simulink model "CLLCTestHarnessPlant"  (R2026a)
settings: Solver=ode23t  StopTime=5e-3  FixedStep=1e-4  MaxStep=1e-6  AbsTol=1e-3
PreLoadFcn:
  | CLLCConverterDefaultInputParameters;
undefined symbols (not defined in the file or in its folder): CLLCCompensator, CLLCController, CLLCDesign, DiscIntNeverNeededParam
libraries: fl_lib x46, nesl_utility x45, ee_lib x35
(part 1 of 4)
Description:
  | Design of LLC Resonant Converter
settings Model: ExtModeTrigDuration=100  Creator=The MathWorks, Inc.  LastModifiedBy=vsolaise
settings SolverCC: MaxConsecutiveMinStep=10
settings DataIOCC: StateSaveName=tmp_raccel_xout  SignalLoggingName=logsoutCLLCConverter  OutputTimes=[0:1.1*3*Voc/(1*2000):1.1*3*Voc/1]
settings OptimizationCC: EfficientMapNaN2IntZero=off
settings HardwareCC: ProdHWDeviceType=Intel->x86-32 (Windows32)  TargetBitPerPointer=64.0  TargetBitPerSizeT=64.0  TargetBitPerPtrDiffT=64.0  TargetLongLongMode=on  TargetIntDivRoundTo=Zero  TargetEndianess=LittleEndian  TargetWordSize=64.0  TargetHWDeviceType=MATLAB Host  ProdEqTarget=off
settings RTWCC: SystemTargetFile=raccel.tlc  TemplateMakefile=raccel_default_tmf  RTWVerbose=off  RTWUseSimCustomCode=on
settings CodeAppCC: GenerateComments=off  MaxIdLength=128.0  SimulinkBlockComments=off
settings RaccelTargetCC: ExtModeTransport=0.0  ExtModeStaticAllocSize=1000000.0  ENABLE_SLEXEC_SSBRIDGE=1.0  RTWCAPIParams=on  RTWCAPIRootIO=on  MultiwordLength=2048.0
settings SimscapeCC: SimscapeNominalValues="[{\"value\":\"1\",\"unit\":\"A\"},{\"value\":\"1\",\"unit\":\"bar\"},{\"value\":\"1\",\"unit\":\"cm^2\"},{\"value\":\"1\",\"unit\":\"cm^3/s\"},{\"value\":\"1\",\"unit\":\"kJ/kg\"},{\"value\":\"1\",\"unit\":\"kW\"},{\"value\":\"1\",\"unit\":\"l\"},{\"value\":\"1\",\"unit\":\"N\"},{\"value\":\"1\",\"unit\":\"N*m\"},{\"value\":\"1\",\"unit\":\"V\"}]"  SimscapeLogName=SimlogCLLCConverter  SimscapeLogLimitData=off  SimscapeLogDataHistory=5000.0

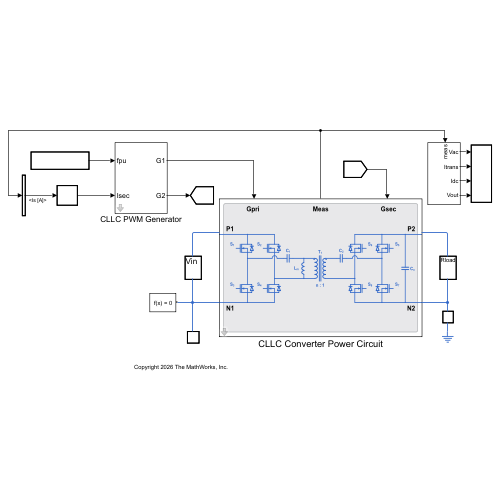
[thumbnail: Simulink's stored preview of the top-level diagram]
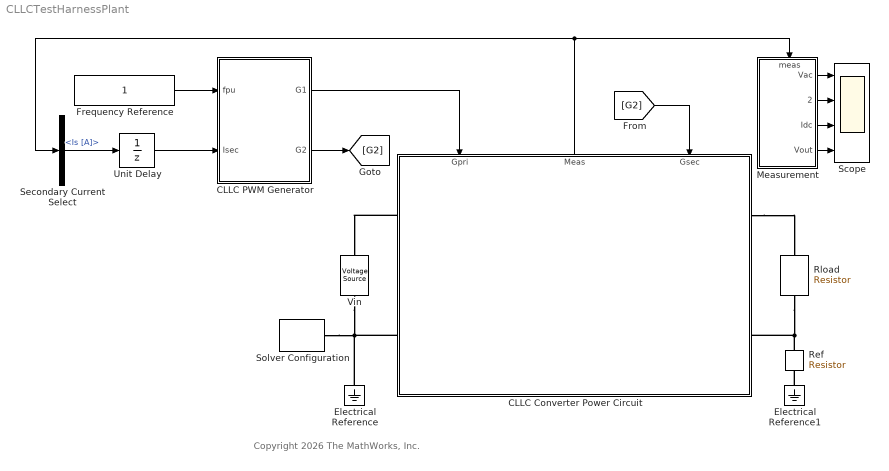
== system CLLCTestHarnessPlant ==
  note: Copyright 2026 The MathWorks, Inc.
  CLLC Converter Power Circuit : Subsystem  mask(CLLC Converter Plant){modelOption=Detailed, C1=6.9269e-7, C1_unit=F, Rcr1=0.001, Rcr1_unit=Ohm, C2=7.487e-7, C2_unit=F, Rcr2=0.001, Rcr2_unit=Ohm, Llk1=3.6568e-6, Llk1_unit=H, R1=0.01, R1_unit=Ohm, Llk2=3.3829e-6, Llk2_unit=H, R2=0.01, R2_unit=Ohm, Lm=5.4852e-5, Lm_unit=H, N1=30, N2=29, Co=1.0667e-3, Co_unit=F, Rco=0.02, Rco_unit=Ohm, Vco=350, Vco_unit=V, PrimaryDeviceOption=Ideal Switch, PrimaryRon=0.0001, PrimaryRon_unit=Ohm, PrimaryGoff=1e-5, PrimaryGoff_unit=1/Ohm, PrimaryVth=2.5, PrimaryVth_unit=V, PrimaryVbodydiodeOn=0.6, PrimaryVbodydiodeOn_unit=V, PrimaryRbodydiodeOn=0.0001, PrimaryRbodydiodeOn_unit=Ohm, PrimaryGbodydiodeOff=1e-5, PrimaryGbodydiodeOff_unit=1/Ohm, PrimaryCparasitic=2e-10, PrimaryCparasitic_unit=F, SecondaryDeviceOption=Ideal Switch, SecondaryRon=0.0001, SecondaryRon_unit=Ohm, SecondaryGoff=1e-5, SecondaryGoff_unit=1/Ohm, SecondaryVth=2.5, SecondaryVth_unit=V, SecondaryVbodydiodeOn=0.6, SecondaryVbodydiodeOn_unit=V, SecondaryRbodydiodeOn=0.0001, SecondaryRbodydiodeOn_unit=Ohm, SecondaryGbodydiodeOff=1e-5, SecondaryGbodydiodeOff_unit=1/Ohm, SecondaryCparasitic=2e-10, SecondaryCparasitic_unit=F, PrimarySimTemp=25, PrimarySimTemp_unit=degC, SecondarySimTemp=25, SecondarySimTemp_unit=degC}
      mask prompts: modelOption "Model option"; C1 "Primary resonant capacitance (C1)"; Rcr1 "Primary resonant capacitor ESR (Rcr1)"; C2 "Secondary resonant capacitance (C2)"; Rcr2 "Secondary resonant capacitor ESR (Rcr2)"; Llk1 "Primary leakage inductance (Llk1)"; R1 "Primary resistance (R1)"; Llk2 "Secondary leakage inductance (Llk2)"; R2 "Secondary resistance (R2)"; Lm "Magnetizing inductance (Lm)"; N1 "Transformer primary number of turns (N1)"; N2 "Transformer secondary number of turns (N2)"; Co "Secondary output capacitance (Co)"; Rco "Secondary output capacitance ESR (Rco)"; Vco "Initial output capacitor voltage"; PrimaryDeviceOption "Select the primary switching device"; PrimaryRon "On-state resistance"; PrimaryGoff "Off-state conductance"; PrimaryVth "Threshold voltage"; PrimaryVbodydiodeOn "Body diode forward voltage"; PrimaryRbodydiodeOn "Body diode on-resistance"; PrimaryGbodydiodeOff "Body diode off-conductance"; PrimaryCparasitic "MOSFET parasitic capacitance"; SecondaryDeviceOption "Select the secondary switching device"; SecondaryRon "On-state resistance"; SecondaryGoff "Off-state conductance"; SecondaryVth "Threshold voltage"; SecondaryVbodydiodeOn "Body diode forward voltage"; SecondaryRbodydiodeOn "Body diode on-resistance"; SecondaryGbodydiodeOff "Body diode off-conductance"; SecondaryCparasitic "MOSFET parasitic capacitance"; PrimarySimTemp "Simulation temperature"; SecondarySimTemp "Simulation temperature"
      mask help: This block models the power circuit of the CLLC resonant converter. You can choose between different semicondcutor switch model for primary and secondaryconverter. You can choose between ideal semiconductor switch, MOSFET without thermal port and tabulated MOSFET with thermal port.
      mask init:
      | %% Unit conversion: convert displayed values to base SI units
      | convMap = containers.Map( ...
      |     {'W','kW','MW','V','kV','mV','F','mF','uF','nF','pF', ...
      |      'H','mH','uH','nH','Ohm','kOhm','mOhm','S','mS','1/Ohm'}, ...
      |     {1, 1e3, 1e6, 1, 1e3, 1e-3, 1, 1e-3, 1e-6, 1e-9, 1e-12, ...
      |      1, 1e-3, 1e-6, 1e-9, 1, 1e3, 1e-3, 1, 1e-3, 1});
      | C1 = C1 * convMap(C1_unit);
      | Rcr1 = Rcr1 * convMap(Rcr1_unit);
      | C2 = C2 * convMap(C2_unit);
      | Rcr2 = Rcr2 * convMap(Rcr2_unit);
      | Llk1 = Llk1 * convMap(Llk1_unit);
      | R1 = R1 * convMap(R1_unit);
      | Llk2 = Llk2 * convMap(Llk2_unit);
      | R2 = R2 * convMap(R2_unit);
      | Lm = Lm * convMap(Lm_unit);
      | Co = Co * convMap(Co_unit);
      | Rco = Rco * convMap(Rco_unit);
      | Vco = Vco * convMap(Vco_unit);
      | PrimaryRon = PrimaryRon * convMap(PrimaryRon_unit);
      | PrimaryGoff = PrimaryGoff * convMap(PrimaryGoff_unit);
      | PrimaryVth = PrimaryVth * convMap(PrimaryVth_unit);
      | PrimaryVbodydiodeOn = PrimaryVbodydiodeOn * convMap(PrimaryVbodydiodeOn_unit);
      | PrimaryRbodydiodeOn = PrimaryRbodydiodeOn * convMap(PrimaryRbodydiodeOn_unit);
      | PrimaryGbodydiodeOff = PrimaryGbodydiodeOff * convMap(PrimaryGbodydiodeOff_unit);
      | PrimaryCparasitic = PrimaryCparasitic * convMap(PrimaryCparasitic_unit);
      | SecondaryRon = SecondaryRon * convMap(SecondaryRon_unit);
      | SecondaryGoff = SecondaryGoff * convMap(SecondaryGoff_unit);
      | SecondaryVth = SecondaryVth * convMap(SecondaryVth_unit);
      | SecondaryVbodydiodeOn = SecondaryVbodydiodeOn * convMap(SecondaryVbodydiodeOn_unit);
      | SecondaryRbodydiodeOn = SecondaryRbodydiodeOn * convMap(SecondaryRbodydiodeOn_unit);
      | SecondaryGbodydiodeOff = SecondaryGbodydiodeOff * convMap(SecondaryGbodydiodeOff_unit);
      | SecondaryCparasitic = SecondaryCparasitic * convMap(SecondaryCparasitic_unit);
      | % Simulation temperature (primary bridge, thermal MOSFETs)
      | % Temperature is an OFFSET unit (K = degC + 273.15), so it cannot use the
      | % multiplicative convMap above; convert it explicitly. PrimarySimTemp_K is read directly
      | % by each primary thermal MOSFET junction-temperature initial target and by every
      | % Temperature Source in the primary bridge.
      | if strcmp(PrimarySimTemp_unit, 'degC')
      |     PrimarySimTemp_K = PrimarySimTemp + 273.15;
      | elseif strcmp(PrimarySimTemp_unit, 'K')
      |     PrimarySimTemp_K = PrimarySimTemp;
      | else
      |     error('CLLC Converter Power Circuit: unrecognized simulation-temperature unit "%s" (expected degC or K).', PrimarySimTemp_unit);
      | end
      | % Simulation temperature (secondary bridge, thermal MOSFETs)
      | % Temperature is an OFFSET unit (K = degC + 273.15), so it cannot use the
      | % multiplicative convMap above; convert it explicitly. SecondarySimTemp_K is read directly
      | % by each secondary thermal MOSFET junction-temperature initial target and by every
      | % Temperature Source in the secondary bridge.
      | if strcmp(SecondarySimTemp_unit, 'degC')
      |     SecondarySimTemp_K = SecondarySimTemp + 273.15;
      | elseif strcmp(SecondarySimTemp_unit, 'K')
      |     SecondarySimTemp_K = SecondarySimTemp;
      | else
      |     error('CLLC Converter Power Circuit: unrecognized simulation-temperature unit "%s" (expected degC or K).', SecondarySimTemp_unit);
      | end
      settings: CopyFcn="set_param(gcbh,\"LinkStatus\",\"none\");"  PortSchema="{\"entries\":[{\"content\":{\"sides\":[{\"content\":{\"connectorIds\":[\"LConn1\",\"LConn2\"]},\"type\":\"ConnectorPlacement.EquallySpacedRectSide\",\"uuid\":\"0e984043-8111-4613-9feb-f4d4d19f792a\"},{\"content\":{\"connectorIds\":[\"RConn1\",\"RConn2\"],\"side\":\"RIGHT\"},\"type\":\"ConnectorPlacement.EquallySpacedRectSide\",\"uuid\":\"aee9207a-aaf7-4114-a348-153041cb19a5\"},{\"content\":{\"connectorIds\":[\"In1\",\"Out1\",\"In2\"],\"side\":\"TOP\"},\"type\":\"ConnectorPlacement.EquallySpacedRectSide\",\"uuid\":\"cf17a722-cb18-4642-bf19-4f4ee8ce3a25\"}]},\"type\":\"ConnectorPlacement.EquallySpacedConnector\",\"uuid\":\"0a50e5d5-a4bf-4817-9816-42fb9bad860d\"}],\"packageUris\":[\"http://schema.mathworks.com/mf0/Connector/R2020b\"],\"version\":\"1.0\"}"
      mask Help: web('CLLCPowerCircuit.html')
      mask TypeOptions modelOption: Simplified | Detailed
      mask Callback modelOption: selectCLLCConverterModelOption(gcb);
      mask TypeOptions C1_unit: F | mF | uF | nF | pF
      mask TypeOptions Rcr1_unit: Ohm | kOhm | mOhm
      mask TypeOptions C2_unit: F | mF | uF | nF | pF
      mask TypeOptions Rcr2_unit: Ohm | kOhm | mOhm
      mask TypeOptions Llk1_unit: H | mH | uH | nH
      mask TypeOptions R1_unit: Ohm | kOhm | mOhm
      mask TypeOptions Llk2_unit: H | mH | uH | nH
      mask TypeOptions R2_unit: Ohm | kOhm | mOhm
      mask TypeOptions Lm_unit: H | mH | uH | nH
      mask TypeOptions Co_unit: F | mF | uF | nF | pF
      mask TypeOptions Rco_unit: Ohm | kOhm | mOhm
      mask TypeOptions Vco_unit: V | kV | mV
      mask TypeOptions PrimaryDeviceOption: Ideal Switch | MOSFET (Ideal, Switching) with Thermal
      mask Callback PrimaryDeviceOption: selectCLLCPrimaryMOSFET(gcb);
      mask TypeOptions PrimaryRon_unit: Ohm | kOhm | mOhm
      mask TypeOptions PrimaryGoff_unit: 1/Ohm | S | mS
      mask TypeOptions PrimaryVth_unit: V | kV | mV
      mask TypeOptions PrimaryVbodydiodeOn_unit: V | mV
      mask TypeOptions PrimaryRbodydiodeOn_unit: Ohm | kOhm | mOhm
      mask TypeOptions PrimaryGbodydiodeOff_unit: 1/Ohm | S | mS
      mask TypeOptions PrimaryCparasitic_unit: F | mF | uF | nF | pF
      mask TypeOptions SecondaryDeviceOption: Ideal Switch | MOSFET (Ideal, Switching) with Thermal
      mask Callback SecondaryDeviceOption: selectCLLCSecondaryMOSFET(gcb);
      mask TypeOptions SecondaryRon_unit: Ohm | kOhm | mOhm
      mask TypeOptions SecondaryGoff_unit: 1/Ohm | S | mS
      mask TypeOptions SecondaryVth_unit: V | kV | mV
      mask TypeOptions SecondaryVbodydiodeOn_unit: V | mV
      mask TypeOptions SecondaryRbodydiodeOn_unit: Ohm | kOhm | mOhm
      mask TypeOptions SecondaryGbodydiodeOff_unit: 1/Ohm | S | mS
      mask TypeOptions SecondaryCparasitic_unit: F | mF | uF | nF | pF
      mask TypeOptions PrimarySimTemp_unit: degC | K
      mask TypeOptions SecondarySimTemp_unit: degC | K
      mask DialogControl ParameterGroupVar Prompt: CLLC Resonant Converter Plant
      mask DialogControl CLLCTank Prompt: CLLC converter parameters
      mask DialogControl TransformerParameters Prompt: Transformer
      mask DialogControl PrimarySwitch Prompt: Primary semiconductor switch
      mask DialogControl PrimaryOpenMOSFETMask Prompt: Open the MOSFET block mask
      mask DialogControl PrimaryOpenMOSFETMask Callback: openCLLCDeviceMask(gcb, 'primaryThermalMOSFET');
      mask DialogControl PrimaryApplyMOSFETParam Prompt: Apply parameters to all primary MOSFET blocks
      mask DialogControl PrimaryApplyMOSFETParam Callback: applyCLLCDeviceParameters(gcb, 'primaryThermalMOSFET');
      mask DialogControl SecondarySwitch Prompt: Secondary semiconductor switch
      mask DialogControl SecondaryOpenMOSFETMask Prompt: Open the MOSFET block mask
      mask DialogControl SecondaryOpenMOSFETMask Callback: openCLLCDeviceMask(gcb, 'secondaryThermalMOSFET');
      mask DialogControl SecondaryApplyMOSFETParam Prompt: Apply parameters to all secondary MOSFET blocks
      mask DialogControl SecondaryApplyMOSFETParam Callback: applyCLLCDeviceParameters(gcb, 'secondaryThermalMOSFET');
      mask DialogControl ExportPanel Prompt: Export to Unmasked Subsystem
      mask DialogControl ExportInfo Prompt: To customize the converter, export it as an unmasked subsystem with the active variant flattened - a standalone, fully-editable circuit plus a parameter file. Requires the "Variant Manager for Simulink" add-on.
      mask DialogControl exportToModel Prompt: Export
      mask DialogControl exportToModel Callback: exportConverterModelFromMask(gcb);
      mask Display: image('CLLCConverterIcon.svg');
  CLLC PWM Generator : Subsystem  mask(CLLC Resonant Converter PWM Generator){solverMode=Variable-step (continuous), Ts=(CLLCController.deadTime/2), Fbase=(CLLCDesign.resonantFreq), fpuMin=(CLLCController.minPUfrequency), fpuMax=(CLLCController.maxPUfrequency*1.3), pulseWidth=0.5, Tdead=(CLLCController.deadTime), Ith=(CLLCCompensator.SRCurrentThreshold), fpuSrLower=0.97, fpuSrUpper=1.03, Tsr=(CLLCController.deadTime), gateVoltageOn=10, gateVoltageOff=0, srGateVoltageOn=10, srGateVoltageOff=0}
      mask prompts: solverMode "Solver mode"; Ts "Sample time (s)"; Fbase "Base (resonant) frequency (Hz)"; fpuMin "Minimum normalized frequency (pu)"; fpuMax "Maximum normalized frequency (pu)"; pulseWidth "Pulse width (fraction of switching period)"; Tdead "Dead time (s)"; Ith "Rectifier current threshold (A)"; fpuSrLower "Resonance band lower edge (pu)"; fpuSrUpper "Resonance band upper edge (pu)"; Tsr "Rectifier turn-on delay (s)"; gateVoltageOn "Gate ON voltage (V)"; gateVoltageOff "Gate OFF voltage (V)"; srGateVoltageOn "Rectifier gate ON voltage (V)"; srGateVoltageOff "Rectifier gate OFF voltage (V)"
      mask help:
      | This block generates full-bridge PWM gate signals with a dead time from a commanded switching frequency, and synchronous rectifier gate signals from the rectifier current.
      |
      | Set the rectifier band lower edge below its upper edge. For a variable-step solver, set Solver mode to Variable-step (continuous). For a fixed-step solver, set Solver mode to Fixed-step (discrete) and set Sample time to a positive value.
      mask init:
      | % Solver mode. Switch every sawtooth ramp in this block between its continuous
      | % and its discrete implementation, and show the sample time only when it is used.
      | pwmGeneratorBlock = gcb;
      | if strcmp(get_param(pwmGeneratorBlock, 'solverMode'), 'Fixed-step (discrete)')
      |     pwmGeneratorRampChoice = 'FixedStep';
      |     pwmGeneratorSampleTimeVisibility = 'on';
      | else
      |     pwmGeneratorRampChoice = 'VariableStep';
      |     pwmGeneratorSampleTimeVisibility = 'off';
      | end
      | 
      | % A block may hold more than one ramp, at any depth, so the ramps are found by the
      | % "Ramp Mode" suffix on their names rather than by one fixed path. The match filter
      | % keeps every variant choice in the search, which is also what silences the
      | % find_system default-variants warning.
      | pwmGeneratorRamps = find_system(pwmGeneratorBlock, ...
      |     'MatchFilter', @Simulink.match.allVariants, 'LookUnderMasks', 'all', ...
      |     'FollowLinks', 'on', 'Regexp', 'on', 'BlockType', 'SubSystem', ...
      |     'Name', 'Ramp Mode$');
      | for pwmGeneratorRampIndex = 1:numel(pwmGeneratorRamps)
      |     set_param(pwmGeneratorRamps{pwmGeneratorRampIndex}, ...
      |         'LabelModeActiveChoice', pwmGeneratorRampChoice);
      | end
      | 
      | % Only the discrete ramp declares a rate, so the sample time is hidden in the
      | % continuous mode. The guard keeps the code silent on a mask still being built.
      | pwmGeneratorMask = Simulink.Mask.get(pwmGeneratorBlock);
      | pwmGeneratorSampleTime = pwmGeneratorMask.getParameter('Ts');
      | if ~isempty(pwmGeneratorSampleTime)
      |     pwmGeneratorSampleTime.Visible = pwmGeneratorSampleTimeVisibility;
      | end
      mask Help: web('CLLCPWMGenerator.html')
      mask TypeOptions solverMode: Variable-step (continuous) | Fixed-step (discrete)
      mask Callback solverMode:
      | % Solver mode. Switch every sawtooth ramp in this block between its continuous
      | % and its discrete implementation, and show the sample time only when it is used.
      | pwmGeneratorBlock = gcb;
      | if strcmp(get_param(pwmGeneratorBlock, 'solverMode'), 'Fixed-step (discrete)')
      |     pwmGeneratorRampChoice = 'FixedStep';
      |     pwmGeneratorSampleTimeVisibility = 'on';
      | else
      |     pwmGeneratorRampChoice = 'VariableStep';
      |     pwmGeneratorSampleTimeVisibility = 'off';
      | end
      | 
      | % A block may hold more than one ramp, at any depth, so the ramps are found by the
      | % "Ramp Mode" suffix on their names rather than by one fixed path. The match filter
      | % keeps every variant choice in the search, which is also what silences the
      | % find_system default-variants warning.
      | pwmGeneratorRamps = find_system(pwmGeneratorBlock, ...
      |     'MatchFilter', @Simulink.match.allVariants, 'LookUnderMasks', 'all', ...
      |     'FollowLinks', 'on', 'Regexp', 'on', 'BlockType', 'SubSystem', ...
      |     'Name', 'Ramp Mode$');
      | for pwmGeneratorRampIndex = 1:numel(pwmGeneratorRamps)
      |     set_param(pwmGeneratorRamps{pwmGeneratorRampIndex}, ...
      |         'LabelModeActiveChoice', pwmGeneratorRampChoice);
      | end
      | 
      | % Only the discrete ramp declares a rate, so the sample time is hidden in the
      | % continuous mode. The guard keeps the code silent on a mask still being built.
      | pwmGeneratorMask = Simulink.Mask.get(pwmGeneratorBlock);
      | pwmGeneratorSampleTime = pwmGeneratorMask.getParameter('Ts');
      | if ~isempty(pwmGeneratorSampleTime)
      |     pwmGeneratorSampleTime.Visible = pwmGeneratorSampleTimeVisibility;
      | end
      mask DialogControl DescTextVar Prompt:
      | This block generates full-bridge PWM gate signals with a dead time from a commanded switching frequency, and synchronous rectifier gate signals from the rectifier current.
      | 
      | Set the rectifier band lower edge below its upper edge. For a variable-step solver, set Solver mode to Variable-step (continuous). For a fixed-step solver, set Solver mode to Fixed-step (discrete) and set Sample time to a positive value.
      mask DialogControl SolverPanel Prompt: Solver Settings
      mask DialogControl SwitchingPanel Prompt: Switching Parameters
      mask DialogControl SyncRectifierPanel Prompt: Synchronous Rectifier
      mask DialogControl GateDrivePanel Prompt: Gate Drive
  Electrical Reference : fl_lib/Electrical/Electrical Elements/Electrical Reference
  Electrical Reference1 : fl_lib/Electrical/Electrical Elements/Electrical Reference
  Frequency Reference : Constant
  Measurement : Subsystem
      settings: PortSchema="{\"entries\":[{\"content\":{\"sides\":[{\"content\":{},\"type\":\"ConnectorPlacement.EquallySpacedRectSide\",\"uuid\":\"b5c92219-bd3b-44a8-8a16-1ea587978409\"},{\"content\":{\"connectorIds\":[\"Out1\",\"Out2\",\"Out3\",\"Out4\"],\"side\":\"RIGHT\"},\"type\":\"ConnectorPlacement.EquallySpacedRectSide\",\"uuid\":\"b58951fa-0a4a-415c-91fc-a01c5851cf7b\"},{\"content\":{\"connectorIds\":[\"In1\"],\"side\":\"TOP\"},\"type\":\"ConnectorPlacement.EquallySpacedRectSide\",\"uuid\":\"5d7f8742-bb02-4261-b191-4137e05aff11\"}]},\"type\":\"ConnectorPlacement.EquallySpacedConnector\",\"uuid\":\"cec0d984-b283-4d36-85e7-6ccc2789e1e2\"}],\"packageUris\":[\"http://schema.mathworks.com/mf0/Connector/R2020b\"],\"version\":\"1.0\"}"
  Ref : fl_lib/Electrical/Electrical Elements/Resistor  R=1e5 Ohm  i_specify=off  i_priority=None  i=0 A  i_nominal_specify=off  i_nominal_value=1  i_nominal_unit=A  v_specify=off  v_priority=None  v=0 V  v_nominal_specify=off  v_nominal_value=1  v_nominal_unit=V
  Rload : fl_lib/Electrical/Electrical Elements/Resistor  R=90 Ohm  i_specify=off  i_priority=None  i=0 A  i_nominal_specify=off  i_nominal_value=1  i_nominal_unit=A  v_specify=off  v_priority=None  v=0 V  v_nominal_specify=off  v_nominal_value=1  v_nominal_unit=V
  Scope : Scope  NumInputPorts=4
      settings: Title=Resonant Tank Voltages  ActiveDisplayYMinimum=-476.51206821820409  ActiveDisplayYMaximum=476.5119903580383
  Secondary Current Select : BusSelector  OutputSignals=ResonantTank.Is [A]
  Solver Configuration : nesl_utility/Solver Configuration  PhysicalDomain=network_engine_domain  SubClassName=solver  LeftPortType=input  RightPortType=generic  Tones=[]  Harmonics=[]  SimulateNoise=off  Profile=off  UseLocalSampling=off  EnableSwitchedLinearOptims=on  FrequencyDomain=off  UseCCode=off  RelTol=0.001  AbsTol=0.001  MinStep=1e-09  ToWorkspace=off  RevertToSquareIcSolve=off  NumHomotopyIterations=100  PhasorMode=off  PhasorModeNumHarmonics=1  ConsistencySolver=NEWTON_XTOL_AFTER_FTOL  CanonicalOrdering=UNORDERED  OptimizeIntermediates=UNOPTIMIZED  IndexReductionMethod=DerivativeReplacement  DoDC=off  ResidualTolerance=1e-09  ConsistencyTolSource=GLOBAL  ConsistencyAbsTol=0.001  ConsistencyRelTol=0.001  ConsistencyTolFactor=0.001  UseLocalSolver=on  LocalSolverChoice=NE_PARTITIONING_ADVANCER  ResolveIndetEquations=off  FunctionEvalNumThread=1  LocalSolverSampleTime=CLLCController.deadTime/3  DoFixedCost=on  MaxNonlinIter=5  MaxModeIter=10  ComputeImpulses=off  ImpulseIterations=2  LinearAlgebra=auto  LinearAlgebraNumThread=0  EquationFormulation=NE_TIME_EF  DelaysMemoryBudget=1024  AutomaticFiltering=on  FilteringTimeConstant=0.001  PartitionStorageMethod=AS_NEEDED  PartitionMemoryBudget=1024  PartitionMethod=ROBUST  MultibodyUseLocalSolver=off  MultibodyLocalSolverChoice=ODE1  MultibodyLocalSolverSampleTime=0.001
  Unit Delay : UnitDelay  SampleTime=-1
  Vin : ee_lib/Sources/Voltage Source  dc_voltage=380 V  ac_voltage=0 V  ac_shift=0 rad  ac_frequency=0 Hz  noise_mode=ee.enum.sources.noise.Disabled  PSD=0 V^2/Hz  sample_time=1e-3 s  repeatability=ee.enum.sources.repeatability.NotRepeatable  user_seed=0  auto_seed=3499211588  i_specify=off  i_priority=None  i=0 A  i_nominal_specify=off  i_nominal_value=1  i_nominal_unit=A  v_specify=off  v_priority=None  v=0 V  v_nominal_specify=off  v_nominal_value=1  v_nominal_unit=V
  wires:
  Measurement/1(Vac) -> Scope/1
  Measurement/2(Itrans) -> Scope/2
  Measurement/3(Idc) -> Scope/3
  Measurement/4(Vout) -> Scope/4
  CLLC Converter Power Circuit/1(Meas) -> Measurement/1(meas), Secondary Current Select/1
  Frequency Reference/1 -> CLLC PWM Generator/1(fpu)
  Secondary Current Select/1 -> Unit Delay/1  "<Is [A]>"
  Unit Delay/1 -> CLLC PWM Generator/2(Isec)
  CLLC PWM Generator/1(G1) -> CLLC Converter Power Circuit/1(Gpri)
  CLLC PWM Generator/2(G2) -> [G2]
  [G2] -> CLLC Converter Power Circuit/2(Gsec)
  connections:
  Vin/RConn1 -- Solver Configuration/RConn1 -- Electrical Reference/LConn1 -- CLLC Converter Power Circuit/LConn2
  Electrical Reference1/LConn1 -- Ref/RConn1
  CLLC Converter Power Circuit/LConn1 -- Vin/LConn1
  CLLC Converter Power Circuit/RConn1 -- Rload/LConn1
  Ref/LConn1 -- Rload/RConn1 -- CLLC Converter Power Circuit/RConn2

== system CLLCTestHarnessPlant/CLLC Converter Power Circuit ==
  Gpri : Inport
  Gsec : Inport  Port=2
  CLLCConverterVariant : Subsystem  Variant=on  VariantControlMode=label  LabelModeActiveChoice=DetailedModel
  P1 : PMIOPort  Side=Left
  N1 : PMIOPort  Port=2  Side=Left
  P2 : PMIOPort  Port=3  Side=Right
  N2 : PMIOPort  Port=4  Side=Right
  Meas : Outport
  wires:
  CLLCConverterVariant/1(Meas) -> Meas/1
  Gsec/1 -> CLLCConverterVariant/2(Gsec)
  Gpri/1 -> CLLCConverterVariant/1(Gpri)
  connections:
  CLLCConverterVariant/RConn2 -- N2/RConn1
  CLLCConverterVariant/RConn1 -- P2/RConn1
  CLLCConverterVariant/LConn2 -- N1/RConn1
  CLLCConverterVariant/LConn1 -- P1/RConn1

== system CLLCTestHarnessPlant/CLLC PWM Generator ==
  fpu : Inport
  Isec : Inport  Port=2
  Frequency Limit : Saturate  UpperLimit=fpuMax  LowerLimit=fpuMin
  Primary Gate Signal : Subsystem
  Synchronous Rectifier : Subsystem
  G1 : Outport
  G2 : Outport  Port=2
  wires:
  Synchronous Rectifier/1(Gs) -> G2/1
  Isec/1 -> Synchronous Rectifier/3(Isec)
  Primary Gate Signal/1(G) -> G1/1
  Primary Gate Signal/2(gates) -> Synchronous Rectifier/1(primaryGates)
  Frequency Limit/1 -> Synchronous Rectifier/2(fpu), Primary Gate Signal/1(fpu)
  fpu/1 -> Frequency Limit/1

== system CLLCTestHarnessPlant/Measurement ==
  BusElementIn5 : Inport  PortName=meas  Element=ResonantTank.Vp [V]
  BusElementIn6 : Inport  PortName=meas  Element=ResonantTank.Ip [A]
  BusElementIn7 : Inport  PortName=meas  Element=ResonantTank.Is [A]
  BusElementIn8 : Inport  PortName=meas  Element=ResonantTank.Vs [A]
  BusElementIn10 : Inport  PortName=meas  Element=Inverter.Iin [A]
  BusElementIn9 : Inport  PortName=meas  Element=Rectifier.Iout [A]
  BusElementIn : Inport  PortName=meas  Element=Rectifier.Vout [V]
  Bus Creator : BusCreator  Inputs=2
  Bus Creator1 : BusCreator  Inputs=2
  Bus Creator2 : BusCreator  Inputs=2
  Vac : Outport
  Itrans : Outport  Port=2
  Idc : Outport  Port=3
  Vout : Outport  Port=4
  wires:
  BusElementIn5/1 -> Bus Creator/1  "Vprimary"
  BusElementIn8/1 -> Bus Creator/2  "Vsecondary"
  BusElementIn10/1 -> Bus Creator2/2  "Iin"
  BusElementIn/1 -> Vout/1  "Vout"
  Bus Creator/1 -> Vac/1
  BusElementIn9/1 -> Bus Creator2/1  "Iout"
  Bus Creator2/1 -> Idc/1
  BusElementIn6/1 -> Bus Creator1/1  "Iprimary"
  BusElementIn7/1 -> Bus Creator1/2  "Isecondary"
  Bus Creator1/1 -> Itrans/1

== system CLLCTestHarnessPlant/CLLC Converter Power Circuit/CLLCConverterVariant ==
  Gpri : Inport
  Gsec : Inport  Port=2
  DetailedModel : Subsystem  VariantControl=DetailedModel
  SimplifiedModel : Subsystem  VariantControl=SimplifiedModel
  P1 : PMIOPort  Side=Left
  P2 : PMIOPort  Port=2  Side=Right
  N1 : PMIOPort  Port=3  Side=Left
  N2 : PMIOPort  Port=4  Side=Right
  Meas : Outport

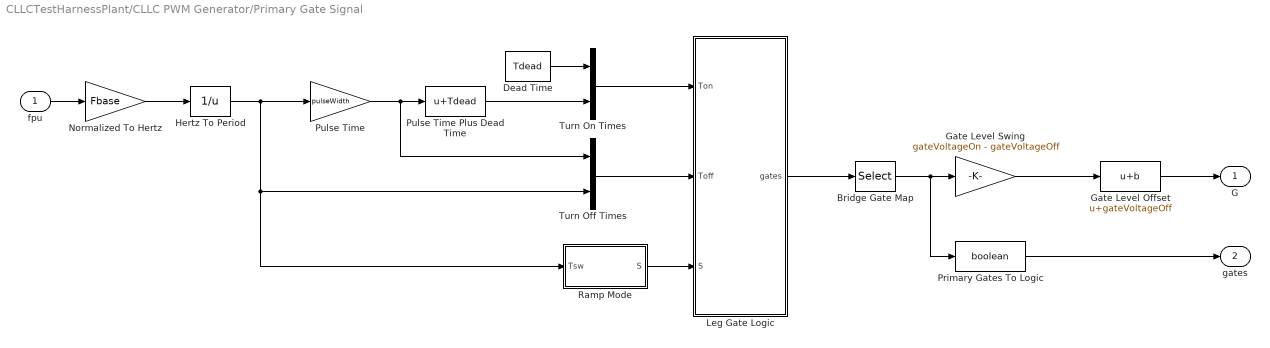
== system CLLCTestHarnessPlant/CLLC PWM Generator/Primary Gate Signal ==
  fpu : Inport
  Bridge Gate Map : Selector  InputPortWidth=2  IndexOptions=Index vector (dialog)  Indices=[1 2 2 1]  OutputSizes=1
  Dead Time : Constant  Value=Tdead
  Gate Level Offset : Bias  Bias=gateVoltageOff
  Gate Level Swing : Gain  Gain=gateVoltageOn - gateVoltageOff
  Hertz To Period : Math  Operator=reciprocal
  Leg Gate Logic : Subsystem
  Normalized To Hertz : Gain  Gain=Fbase
  Primary Gates To Logic : DataTypeConversion  OutDataTypeStr=boolean
  Pulse Time : Gain  Gain=pulseWidth
  Pulse Time Plus Dead Time : Bias  Bias=Tdead
  Ramp Mode : Subsystem  Variant=on  VariantControlMode=label  LabelModeActiveChoice=VariableStep
  Turn Off Times : Mux  Inputs=2
  Turn On Times : Mux  Inputs=2
  G : Outport
  gates : Outport  Port=2
  wires:
  Primary Gates To Logic/1 -> gates/1
  Gate Level Offset/1 -> G/1
  Bridge Gate Map/1 -> Primary Gates To Logic/1, Gate Level Swing/1
  Leg Gate Logic/1(gates) -> Bridge Gate Map/1
  Ramp Mode/1(S) -> Leg Gate Logic/3(S)
  Turn Off Times/1 -> Leg Gate Logic/2(Toff)
  Turn On Times/1 -> Leg Gate Logic/1(Ton)
  Pulse Time Plus Dead Time/1 -> Turn On Times/2
  Dead Time/1 -> Turn On Times/1
  Pulse Time/1 -> Turn Off Times/1, Pulse Time Plus Dead Time/1
  Hertz To Period/1 -> Ramp Mode/1(Tsw), Turn Off Times/2, Pulse Time/1
  Normalized To Hertz/1 -> Hertz To Period/1
  fpu/1 -> Normalized To Hertz/1
  Gate Level Swing/1 -> Gate Level Offset/1

== system CLLCTestHarnessPlant/CLLC PWM Generator/Synchronous Rectifier ==
  primaryGates : Inport
  fpu : Inport  Port=2
  Isec : Inport  Port=3
  Conduction Detect : Subsystem
  Rectifier Gate Level Offset : Bias  Bias=srGateVoltageOff
  Rectifier Gate Level Swing : Gain  Gain=srGateVoltageOn - srGateVoltageOff
  Rectifier Gates To Double : DataTypeConversion  OutDataTypeStr=double
  Region Select : Subsystem
  Turn On Delay : Subsystem
  Gs : Outport
  wires:
  Rectifier Gate Level Offset/1 -> Gs/1
  Rectifier Gates To Double/1 -> Rectifier Gate Level Swing/1
  Turn On Delay/1(Gs) -> Rectifier Gates To Double/1
  Region Select/1(Gs) -> Turn On Delay/1(condition)
  Conduction Detect/1(permit) -> Region Select/3(permit)
  Isec/1 -> Conduction Detect/1(Isec)
  fpu/1 -> Region Select/2(fpu)
  primaryGates/1 -> Region Select/1(primaryGates)
  Rectifier Gate Level Swing/1 -> Rectifier Gate Level Offset/1

== system CLLCTestHarnessPlant/CLLC Converter Power Circuit/CLLCConverterVariant/DetailedModel ==
  Gpri : Inport
  Gsec : Inport  Port=2
  Bus Creator : BusCreator  Inputs=3
  Primary Converter : Subsystem
      settings: PortSchema="{\"entries\":[{\"content\":{\"sides\":[{\"content\":{\"connectorIds\":[\"LConn1\",\"LConn2\"]},\"type\":\"ConnectorPlacement.EquallySpacedRectSide\",\"uuid\":\"5f98eff0-54e4-47a8-aeeb-0279cba14f26\"},{\"content\":{\"connectorIds\":[\"RConn1\",\"RConn2\"],\"side\":\"RIGHT\"},\"type\":\"ConnectorPlacement.EquallySpacedRectSide\",\"uuid\":\"71acbbb6-1fc8-426c-b389-5d494eb18bfd\"},{\"content\":{\"connectorIds\":[\"In1\",\"Out1\"],\"side\":\"TOP\"},\"type\":\"ConnectorPlacement.EquallySpacedRectSide\",\"uuid\":\"dc77ee05-1f57-4323-bfda-b0076e2d1ee5\"}]},\"type\":\"ConnectorPlacement.EquallySpacedConnector\",\"uuid\":\"8d0b8c05-d5c5-4033-af60-ebdb639bdc40\"}],\"packageUris\":[\"http://schema.mathworks.com/mf0/Connector/R2020b\"],\"version\":\"1.0\"}"
  Resonant Tank : Subsystem
      settings: PortSchema="{\"entries\":[{\"content\":{\"sides\":[{\"content\":{\"connectorIds\":[\"LConn1\",\"LConn2\"]},\"type\":\"ConnectorPlacement.EquallySpacedRectSide\",\"uuid\":\"d505f362-3b8e-4dee-9b5b-731d75550efb\"},{\"content\":{\"connectorIds\":[\"RConn1\",\"RConn2\"],\"side\":\"RIGHT\"},\"type\":\"ConnectorPlacement.EquallySpacedRectSide\",\"uuid\":\"66ab4b84-9b7a-404b-b3f6-3ac1c371ea42\"},{\"content\":{\"connectorIds\":[\"Out1\"],\"side\":\"TOP\"},\"type\":\"ConnectorPlacement.EquallySpacedRectSide\",\"uuid\":\"00605859-d490-4a3b-aace-391362dfba7e\"}]},\"type\":\"ConnectorPlacement.EquallySpacedConnector\",\"uuid\":\"a210fe68-7181-499f-8e1c-ccfe71b42a4c\"}],\"packageUris\":[\"http://schema.mathworks.com/mf0/Connector/R2020b\"],\"version\":\"1.0\"}"
      mask Display: image('CLLCTransformerIcon.png');
  Secondary Converter : Subsystem
      settings: PortSchema="{\"entries\":[{\"content\":{\"sides\":[{\"content\":{\"connectorIds\":[\"LConn1\",\"LConn2\"]},\"type\":\"ConnectorPlacement.EquallySpacedRectSide\",\"uuid\":\"4786b3cc-2245-4c72-a50b-9c63e4ad3d8a\"},{\"content\":{\"connectorIds\":[\"RConn1\",\"RConn2\"],\"side\":\"RIGHT\"},\"type\":\"ConnectorPlacement.EquallySpacedRectSide\",\"uuid\":\"250a01d0-bf95-4e01-bf69-d866bcf3b7bd\"},{\"content\":{\"connectorIds\":[\"In1\",\"Out1\"],\"side\":\"TOP\"},\"type\":\"ConnectorPlacement.EquallySpacedRectSide\",\"uuid\":\"52730d18-084b-4644-8b2a-b54c84fa88ec\"}]},\"type\":\"ConnectorPlacement.EquallySpacedConnector\",\"uuid\":\"d24cae2a-f132-4f5a-ac35-d7440d7a99e9\"}],\"packageUris\":[\"http://schema.mathworks.com/mf0/Connector/R2020b\"],\"version\":\"1.0\"}"
  P1 : PMIOPort  Side=Left
  P2 : PMIOPort  Port=2  Side=Right
  N1 : PMIOPort  Port=3  Side=Left
  N2 : PMIOPort  Port=4  Side=Right
  Meas : Outport
  wires:
  Gpri/1 -> Primary Converter/1(G)
  Gsec/1 -> Secondary Converter/1(G)
  Primary Converter/1(meas) -> Bus Creator/1  "Inverter"
  Secondary Converter/1(meas) -> Bus Creator/3  "Rectifier"
  Bus Creator/1 -> Meas/1
  Resonant Tank/1(meas) -> Bus Creator/2  "ResonantTank"
  connections:
  N1/RConn1 -- Primary Converter/LConn2
  N2/RConn1 -- Secondary Converter/RConn2
  Resonant Tank/LConn1 -- Primary Converter/RConn1
  Resonant Tank/RConn2 -- Secondary Converter/LConn2
  P1/RConn1 -- Primary Converter/LConn1
  P2/RConn1 -- Secondary Converter/RConn1
  Resonant Tank/LConn2 -- Primary Converter/RConn2
  Resonant Tank/RConn1 -- Secondary Converter/LConn1

== system CLLCTestHarnessPlant/CLLC Converter Power Circuit/CLLCConverterVariant/SimplifiedModel ==
  Gpri : Inport
  Gsec : Inport  Port=2
  Bus Creator : BusCreator  Inputs=3
  Primary Converter : Subsystem
      settings: PortSchema="{\"entries\":[{\"content\":{\"sides\":[{\"content\":{\"connectorIds\":[\"LConn1\",\"LConn2\"]},\"type\":\"ConnectorPlacement.EquallySpacedRectSide\",\"uuid\":\"5f98eff0-54e4-47a8-aeeb-0279cba14f26\"},{\"content\":{\"connectorIds\":[\"RConn1\",\"RConn2\"],\"side\":\"RIGHT\"},\"type\":\"ConnectorPlacement.EquallySpacedRectSide\",\"uuid\":\"71acbbb6-1fc8-426c-b389-5d494eb18bfd\"},{\"content\":{\"connectorIds\":[\"In1\",\"Out1\"],\"side\":\"TOP\"},\"type\":\"ConnectorPlacement.EquallySpacedRectSide\",\"uuid\":\"dc77ee05-1f57-4323-bfda-b0076e2d1ee5\"}]},\"type\":\"ConnectorPlacement.EquallySpacedConnector\",\"uuid\":\"8d0b8c05-d5c5-4033-af60-ebdb639bdc40\"}],\"packageUris\":[\"http://schema.mathworks.com/mf0/Connector/R2020b\"],\"version\":\"1.0\"}"
  Resonant Tank : Subsystem
      settings: PortSchema="{\"entries\":[{\"content\":{\"sides\":[{\"content\":{\"connectorIds\":[\"LConn1\",\"LConn2\"]},\"type\":\"ConnectorPlacement.EquallySpacedRectSide\",\"uuid\":\"d505f362-3b8e-4dee-9b5b-731d75550efb\"},{\"content\":{\"connectorIds\":[\"RConn1\",\"RConn2\"],\"side\":\"RIGHT\"},\"type\":\"ConnectorPlacement.EquallySpacedRectSide\",\"uuid\":\"66ab4b84-9b7a-404b-b3f6-3ac1c371ea42\"},{\"content\":{\"connectorIds\":[\"Out1\"],\"side\":\"TOP\"},\"type\":\"ConnectorPlacement.EquallySpacedRectSide\",\"uuid\":\"00605859-d490-4a3b-aace-391362dfba7e\"}]},\"type\":\"ConnectorPlacement.EquallySpacedConnector\",\"uuid\":\"a210fe68-7181-499f-8e1c-ccfe71b42a4c\"}],\"packageUris\":[\"http://schema.mathworks.com/mf0/Connector/R2020b\"],\"version\":\"1.0\"}"
      mask Display: image('CLLCTransformerIcon.png');
  Secondary Converter : Subsystem
      settings: PortSchema="{\"entries\":[{\"content\":{\"sides\":[{\"content\":{\"connectorIds\":[\"LConn1\",\"LConn2\"]},\"type\":\"ConnectorPlacement.EquallySpacedRectSide\",\"uuid\":\"4786b3cc-2245-4c72-a50b-9c63e4ad3d8a\"},{\"content\":{\"connectorIds\":[\"RConn1\",\"RConn2\"],\"side\":\"RIGHT\"},\"type\":\"ConnectorPlacement.EquallySpacedRectSide\",\"uuid\":\"250a01d0-bf95-4e01-bf69-d866bcf3b7bd\"},{\"content\":{\"connectorIds\":[\"In1\",\"Out1\"],\"side\":\"TOP\"},\"type\":\"ConnectorPlacement.EquallySpacedRectSide\",\"uuid\":\"52730d18-084b-4644-8b2a-b54c84fa88ec\"}]},\"type\":\"ConnectorPlacement.EquallySpacedConnector\",\"uuid\":\"d24cae2a-f132-4f5a-ac35-d7440d7a99e9\"}],\"packageUris\":[\"http://schema.mathworks.com/mf0/Connector/R2020b\"],\"version\":\"1.0\"}"
  P1 : PMIOPort  Side=Left
  P2 : PMIOPort  Port=2  Side=Right
  N1 : PMIOPort  Port=3  Side=Left
  N2 : PMIOPort  Port=4  Side=Right
  Meas : Outport
  wires:
  Resonant Tank/1(meas) -> Bus Creator/2  "ResonantTank"
  Bus Creator/1 -> Meas/1
  Secondary Converter/1(meas) -> Bus Creator/3  "Rectifier"
  Primary Converter/1(meas) -> Bus Creator/1  "Inverter"
  Gsec/1 -> Secondary Converter/1(G)
  Gpri/1 -> Primary Converter/1(G)
  connections:
  Resonant Tank/RConn1 -- Secondary Converter/LConn1
  Resonant Tank/LConn2 -- Primary Converter/RConn2
  P2/RConn1 -- Secondary Converter/RConn1
  P1/RConn1 -- Primary Converter/LConn1
  Resonant Tank/RConn2 -- Secondary Converter/LConn2
  Resonant Tank/LConn1 -- Primary Converter/RConn1
  N2/RConn1 -- Secondary Converter/RConn2
  N1/RConn1 -- Primary Converter/LConn2

== system CLLCTestHarnessPlant/CLLC PWM Generator/Primary Gate Signal/Leg Gate Logic ==
  Ton : Inport
  Toff : Inport  Port=2
  S : Inport  Port=3
  After Turn Off : RelationalOperator
  After Turn On : RelationalOperator
  Pulse Window : Logic  Operator=XOR
  To Double : DataTypeConversion  OutDataTypeStr=double
  gates : Outport
  wires:
  To Double/1 -> gates/1
  Pulse Window/1 -> To Double/1
  After Turn Off/1 -> Pulse Window/2
  After Turn On/1 -> Pulse Window/1
  S/1 -> After Turn On/1, After Turn Off/1
  Toff/1 -> After Turn Off/2
  Ton/1 -> After Turn On/2

== system CLLCTestHarnessPlant/CLLC PWM Generator/Primary Gate Signal/Ramp Mode ==
  Tsw : Inport
  FixedStep : Subsystem  VariantControl=FixedStep
  VariableStep : Subsystem  VariantControl=VariableStep
  S : Outport

== system CLLCTestHarnessPlant/CLLC PWM Generator/Synchronous Rectifier/Conduction Detect ==
  Isec : Inport
  Conduction Pair : Mux  Inputs=2
  Forward Conduction : RelationalOperator
  Forward Threshold : Constant  Value=Ith
  Rectifier Gate Map : Selector  InputPortWidth=2  IndexOptions=Index vector (dialog)  Indices=[1 2 2 1]  OutputSizes=1
  Reverse Conduction : RelationalOperator  Operator=<=
  Reverse Threshold : Constant  Value=-Ith
  permit : Outport
  wires:
  Rectifier Gate Map/1 -> permit/1
  Conduction Pair/1 -> Rectifier Gate Map/1
  Reverse Conduction/1 -> Conduction Pair/2
  Forward Conduction/1 -> Conduction Pair/1
  Reverse Threshold/1 -> Reverse Conduction/2
  Forward Threshold/1 -> Forward Conduction/2
  Isec/1 -> Reverse Conduction/1, Forward Conduction/1

== system CLLCTestHarnessPlant/CLLC PWM Generator/Synchronous Rectifier/Region Select ==
  primaryGates : Inport
  fpu : Inport  Port=2
  permit : Inport  Port=3
  Above Resonance : Subsystem
  Below Resonance : Subsystem
  If : If  IfExpression=u1 <= fpuSrLower  ElseIfExpressions=u1 >= fpuSrUpper  SampleTime=0
  Rectifier Gates : Merge  Inputs=3
  Within Band : Subsystem
  Gs : Outport
  wires:
  Rectifier Gates/1 -> Gs/1
  Within Band/1(Gs) -> Rectifier Gates/3
  If/3 -> Within Band/Action
  Above Resonance/1(Gs) -> Rectifier Gates/2
  If/2 -> Above Resonance/Action
  Below Resonance/1(Gs) -> Rectifier Gates/1
  permit/1 -> Within Band/2(permit), Above Resonance/2(permit), Below Resonance/2(permit)
  primaryGates/1 -> Within Band/1(primaryGates), Above Resonance/1(primaryGates), Below Resonance/1(primaryGates)
  If/1 -> Below Resonance/Action
  fpu/1 -> If/1

== system CLLCTestHarnessPlant/CLLC PWM Generator/Synchronous Rectifier/Turn On Delay ==
  condition : Inport
  Delay Elapsed : RelationalOperator
  Delay Time : Constant  Value=Tsr
  Logic To Double : DataTypeConversion  OutDataTypeStr=double
  Rate Offset : Bias  Bias=-1
  Rate Swing : Gain  Gain=2
  Rectifier Gate Window : Logic
  Rectifier Ramp Mode : Subsystem  Variant=on  VariantControlMode=label  LabelModeActiveChoice=VariableStep
  Gs : Outport
  wires:
  Rectifier Gate Window/1 -> Gs/1
  Delay Elapsed/1 -> Rectifier Gate Window/2
  Delay Time/1 -> Delay Elapsed/2
  Rectifier Ramp Mode/1(S) -> Delay Elapsed/1
  Rate Offset/1 -> Rectifier Ramp Mode/1(rate)
  Rate Swing/1 -> Rate Offset/1
  Logic To Double/1 -> Rate Swing/1
  condition/1 -> Rectifier Gate Window/1, Logic To Double/1

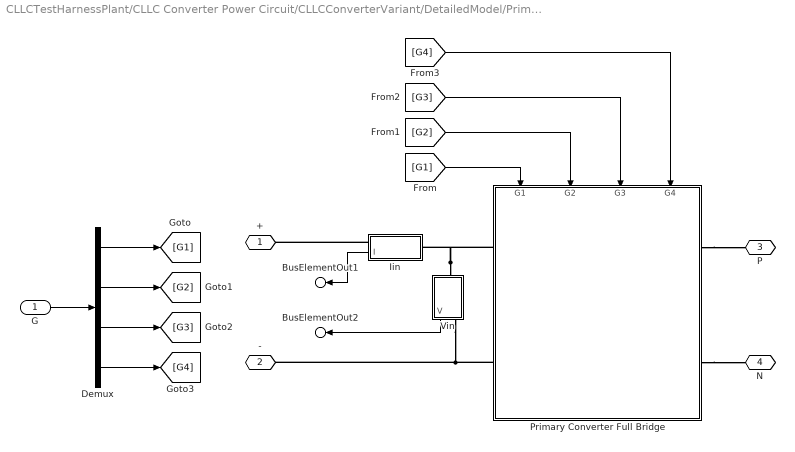
== system CLLCTestHarnessPlant/CLLC Converter Power Circuit/CLLCConverterVariant/DetailedModel/Primary Converter ==
  G : Inport
  Demux : Demux
  Iin : Subsystem
      settings: PortSchema="{\"entries\":[{\"content\":{\"sides\":[{\"content\":{\"connectorIds\":[\"LConn1\",\"Out1\"]},\"type\":\"ConnectorPlacement.EquallySpacedRectSide\",\"uuid\":\"e749c2ff-fd60-426f-a769-b61a7dfe80d2\"},{\"content\":{\"connectorIds\":[\"RConn1\"],\"side\":\"RIGHT\"},\"type\":\"ConnectorPlacement.EquallySpacedRectSide\",\"uuid\":\"f3bb02bd-f8d2-4326-b68c-6f969fa4ac22\"},{\"content\":{\"side\":\"TOP\"},\"type\":\"ConnectorPlacement.EquallySpacedRectSide\",\"uuid\":\"9ab7a0d1-20d8-49e4-8eb3-54d34434204c\"}]},\"type\":\"ConnectorPlacement.EquallySpacedConnector\",\"uuid\":\"19e2a6d5-13f4-47de-bb59-b826817cba83\"}],\"packageUris\":[\"http://schema.mathworks.com/mf0/Connector/R2020b\"],\"version\":\"1.0\"}"
      mask Display: disp("I")
  Primary Converter Full Bridge : Subsystem  Variant=on  VariantControlMode=label  LabelModeActiveChoice=IdealSwitch
      settings: PortSchema="{\"entries\":[{\"content\":{\"sides\":[{\"content\":{\"connectorIds\":[\"LConn1\",\"LConn2\"]},\"type\":\"ConnectorPlacement.EquallySpacedRectSide\",\"uuid\":\"27c41940-d662-4779-afdd-48b642f77411\"},{\"content\":{\"connectorIds\":[\"RConn1\",\"RConn2\"],\"side\":\"RIGHT\"},\"type\":\"ConnectorPlacement.EquallySpacedRectSide\",\"uuid\":\"b0072b01-add1-4b0f-b94e-e1b6c9886b0e\"},{\"content\":{\"connectorIds\":[\"In1\",\"In2\",\"In3\",\"In4\"],\"side\":\"TOP\"},\"type\":\"ConnectorPlacement.EquallySpacedRectSide\",\"uuid\":\"c43bed80-422d-49db-9596-8b38d5c3e411\"},{\"content\":{\"side\":\"BOTTOM\"},\"type\":\"ConnectorPlacement.EquallySpacedRectSide\",\"uuid\":\"01f06046-f57e-45b0-bca5-368a5a543f97\"}]},\"type\":\"ConnectorPlacement.EquallySpacedConnector\",\"uuid\":\"2fcb5370-6bd7-4702-bf87-ebedbb7e376c\"}],\"packageUris\":[\"http://schema.mathworks.com/mf0/Connector/R2020b\"],\"version\":\"1.0\"}"
  Vin : Subsystem
      mask Display: disp("V")
  + : PMIOPort  Side=Left
  - : PMIOPort  Port=2  Side=Left
  P : PMIOPort  Port=3  Side=Right
  N : PMIOPort  Port=4  Side=Right
  BusElementOut2 : Outport  PortName=meas  Element=Vin [V]
  BusElementOut1 : Outport  PortName=meas  Element=Iin [A]
  wires:
  Iin/1(I) -> BusElementOut1/1
  Vin/1(V) -> BusElementOut2/1
  Demux/4 -> [G4]
  Demux/3 -> [G3]
  Demux/2 -> [G2]
  Demux/1 -> [G1]
  G/1 -> Demux/1
  [G1] -> Primary Converter Full Bridge/1(G1)
  [G2] -> Primary Converter Full Bridge/2(G2)
  [G3] -> Primary Converter Full Bridge/3(G3)
  [G4] -> Primary Converter Full Bridge/4(G4)
  connections:
  Iin/LConn1 -- +/RConn1
  Vin/LConn1 -- Iin/RConn1 -- Primary Converter Full Bridge/LConn1
  Vin/RConn1 -- -/RConn1 -- Primary Converter Full Bridge/LConn2
  Primary Converter Full Bridge/RConn1 -- P/RConn1
  Primary Converter Full Bridge/RConn2 -- N/RConn1

== system CLLCTestHarnessPlant/CLLC Converter Power Circuit/CLLCConverterVariant/DetailedModel/Resonant Tank ==
  C1 : fl_lib/Electrical/Electrical Elements/Capacitor  c=C1 F  r=Rcr1 Ohm  g=0 1/Ohm  i_specify=off  i_priority=None  i=0 A  i_nominal_specify=off  i_nominal_value=1  i_nominal_unit=A  v_specify=off  v_priority=None  v=0 V  v_nominal_specify=off  v_nominal_value=1  v_nominal_unit=V  vc_specify=off  vc_priority=None  vc=0 V  vc_nominal_specify=off  vc_nominal_value=1  vc_nominal_unit=V
  C2 : fl_lib/Electrical/Electrical Elements/Capacitor  c=C2 F  r=Rcr2 Ohm  g=0 1/Ohm  i_specify=off  i_priority=None  i=0 A  i_nominal_specify=off  i_nominal_value=1  i_nominal_unit=A  v_specify=off  v_priority=None  v=0 V  v_nominal_specify=off  v_nominal_value=1  v_nominal_unit=V  vc_specify=off  vc_priority=None  vc=0 V  vc_nominal_specify=off  vc_nominal_value=1  vc_nominal_unit=V
  Ip : Subsystem
      settings: PortSchema="{\"entries\":[{\"content\":{\"sides\":[{\"content\":{\"connectorIds\":[\"Out1\",\"LConn1\"]},\"type\":\"ConnectorPlacement.EquallySpacedRectSide\",\"uuid\":\"e749c2ff-fd60-426f-a769-b61a7dfe80d2\"},{\"content\":{\"connectorIds\":[\"RConn1\"],\"side\":\"RIGHT\"},\"type\":\"ConnectorPlacement.EquallySpacedRectSide\",\"uuid\":\"f3bb02bd-f8d2-4326-b68c-6f969fa4ac22\"},{\"content\":{\"side\":\"TOP\"},\"type\":\"ConnectorPlacement.EquallySpacedRectSide\",\"uuid\":\"9ab7a0d1-20d8-49e4-8eb3-54d34434204c\"}]},\"type\":\"ConnectorPlacement.EquallySpacedConnector\",\"uuid\":\"19e2a6d5-13f4-47de-bb59-b826817cba83\"}],\"packageUris\":[\"http://schema.mathworks.com/mf0/Connector/R2020b\"],\"version\":\"1.0\"}"
      mask Display: disp("I")
  Is : Subsystem
      settings: PortSchema="{\"entries\":[{\"content\":{\"sides\":[{\"content\":{\"connectorIds\":[\"LConn1\"]},\"type\":\"ConnectorPlacement.EquallySpacedRectSide\",\"uuid\":\"e749c2ff-fd60-426f-a769-b61a7dfe80d2\"},{\"content\":{\"connectorIds\":[\"RConn1\",\"Out1\"],\"side\":\"RIGHT\"},\"type\":\"ConnectorPlacement.EquallySpacedRectSide\",\"uuid\":\"f3bb02bd-f8d2-4326-b68c-6f969fa4ac22\"},{\"content\":{\"side\":\"TOP\"},\"type\":\"ConnectorPlacement.EquallySpacedRectSide\",\"uuid\":\"9ab7a0d1-20d8-49e4-8eb3-54d34434204c\"}]},\"type\":\"ConnectorPlacement.EquallySpacedConnector\",\"uuid\":\"19e2a6d5-13f4-47de-bb59-b826817cba83\"}],\"packageUris\":[\"http://schema.mathworks.com/mf0/Connector/R2020b\"],\"version\":\"1.0\"}"
      mask Display: disp("I")
  Resonant Transformer : ee_lib/Passive/Transformers/Nonlinear Transformer  Nw=N1  Nw2=N2  winding_param_option=2  Req=0.01 Ohm  Leq=0.0001 H  R_1=R1 Ohm  L_1=Llk1 H  R_2=R2 Ohm  L_2=Llk2 H  averaging_period=0 s  R_m=10000 Ohm  parameterization_option=1  H_data=[0, 200, 400, 600, 800, 1000] A/m  B_data=[0, .81, 1.25, 1.42, 1.48, 1.49] T  length_effective=0.2 m  area_effective=2e-4 m^2  L=Lm H  L_sat=1e-2 H  current_data=[0, .4, .8, 1.2, 1.6, 2] A  magnetic_flux_data=[0, .161, .25, .284, .295, .299] .* 1e-3 Wb  magnetic_flux_sat=1.6e-04 Wb  dBdH0=0.005 T*m/A  B1=1.49 T  H1=1000 A/m  c=0.1  K=200 A/m  alpha=1e-4  interpolation_option=1  Leq_i0=0 A  L1_i0=0 A  L2_i0=0 A  x0_option=1  i_L0=0 A  phi0=0 Wb  B0=0 T  H0=0 A/m  Leq_g=1e-9 1/Ohm  L1_g=0 1/Ohm  L2_g=0 1/Ohm
  Vp : Subsystem
      mask Display: disp("V")
  Vs : Subsystem
      mask Display: disp("V")
  P1 : PMIOPort  Side=Left
  N1 : PMIOPort  Port=2  Side=Left
  P2 : PMIOPort  Port=3  Side=Right
  N2 : PMIOPort  Port=4  Side=Right
  Out Bus Element1 : Outport  PortName=meas  Element=Ip [A]
  Out Bus Element2 : Outport  PortName=meas  Element=Vp [V]
  Out Bus Element3 : Outport  PortName=meas  Element=Is [A]
  Out Bus Element4 : Outport  PortName=meas  Element=Vs [A]
  wires:
  Is/1(I) -> Out Bus Element3/1
  Vp/1(V) -> Out Bus Element2/1
  Ip/1(I) -> Out Bus Element1/1
  Vs/1(V) -> Out Bus Element4/1
  connections:
  C2/RConn1 -- Is/LConn1
  Resonant Transformer/RConn1 -- C2/LConn1
  Resonant Transformer/LConn1 -- C1/RConn1
  Ip/RConn1 -- C1/LConn1
  Vp/RConn1 -- N1/RConn1 -- Resonant Transformer/LConn2
  Vs/RConn1 -- Resonant Transformer/RConn2 -- N2/RConn1
  Vs/LConn1 -- Is/RConn1 -- P2/RConn1
  P1/RConn1 -- Vp/LConn1 -- Ip/LConn1
